simulink model "HFISaliencyTest"  (R2026b)
settings: Solver=ode4  StopTime=hfiTestCfg.Duration  FixedStep=hfiTestCfg.PlantStep
PostLoadFcn:
  | addpath(fullfile(fileparts(get_param(bdroot,'FileName')),'..','build_process'));initialize_hfi_probe_test(bdroot);
model workspace (MAT data in the model file):
  hfPlantCfg.Rs = 0.5
  hfPlantCfg.Ld = 0.001
  hfPlantCfg.Lq = 0.0015
  hfPlantCfg.Flux = 0.035
  hfPlantCfg.PolePairs = 4
  hfPlantCfg.J = 0.0005
  hfPlantCfg.B = 0.0001
  hfPlantCfg.Id0 = 0
  hfPlantCfg.Iq0 = 0
  hfPlantCfg.Speed0 = 0
  hfPlantCfg.Position0 = 0.175
  hfPlantCfg.SaturationDepth = 0
  hfPlantCfg.SaturationCurrent = 1
  hfPlantCfg.CrossInductance = 0
  hfPlantCfg.MechanicalEnabled = 1
  hfPlantCfg.Settings = [0.5; 0.001; 0.0015; 0.035; 4; 0.0005; 0.0001; 0; 1; 0; 1]
  hfPlantCfg.InitialState = [0; 0; 0; 0.175]
  hfiTestCfg.Duration = 0.05
  hfiTestCfg.Ts = 5e-05
  hfiTestCfg.PlantStep = 2.5e-06
  hfiTestCfg.InitialElectricalAngle = 0.7
  hfiTestCfg.InjectionScale = 1
  hfiTestCfg.Enable = 1
  hfiTestCfg.Reset = 0
  hfiTestCfg.LoadTorque = 0
  hfiTestCfg.MeasurementNoise = 0
  hfiTestCfg.NoiseSeed = 42
  hfiTestCfg.CurrentOffset = [0; 0; 0]
  hfiTestCfg.CurrentResolution = 0
  hfiTestCfg.CurrentRange = 8
  hfiTestCfg.CurrentDelay = 0
  hfiTestCfg.VoltageAlignmentDelay = 0
  hfiTestCfg.ExecutionDelay = 0
  hfiTestCfg.ActuationGain = 1
  hfiTestCfg.SaturationDepth = 0
  hfiTestCfg.CrossInductance = 0
  hfiTestCfg.MechanicalEnabled = 1
  probeCfg.Ts = 5e-05
  probeCfg.InjectionVoltage = 5
  probeCfg.WarmupSamples = 32
  probeCfg.CaptureSamples = 256
  probeCfg.MinSaliencyRatio = 0.08
  probeCfg.MaxSaliencyRatio = 0.8
  probeCfg.MinInverseInductance = 100
  probeCfg.MaxInverseInductance = 5000
  probeCfg.MaxFitResidual = 0.2
  probeCfg.MaxAsymmetry = 0.1
  probeCfg.MinVoltageRms = 1
  probeCfg.MaxCurrent = 2
  probeCfg.ProbeAxis = 0
  probeCfg.CrossPhase = 0
  probeCfg.Settings = [5e-05; 5; 32; 256; 0.08; 0.8; 100; 5000; 0.2; 0.1; 1; 2; 0; 0]
  probeCfg.InitialState = [0; 0; 0; 0; 0; 0; 0; 0; 0; 0; 0; 0; 0; 0; 0; 0; 0; 0; 0]
  testStim.time = [0 5e-05 0.0001 0.00015 0.0002 0.00025 0.0003 0.00035 0.0004 0.00045 0.0005 0.00055 ... (1001 elements, 1001x1)]
  testStim.signals.values = [0 0 0 0 0 0 0 0 0 0 0 0 ... (7007 elements, 1001x7)]
  testStim.signals.dimensions = 7
libraries: ClarkePark x2, PMSMHighFrequencyPlant x1, HighFrequencyObserver x1
settings Model: Creator=24322  LastModifiedBy=24322

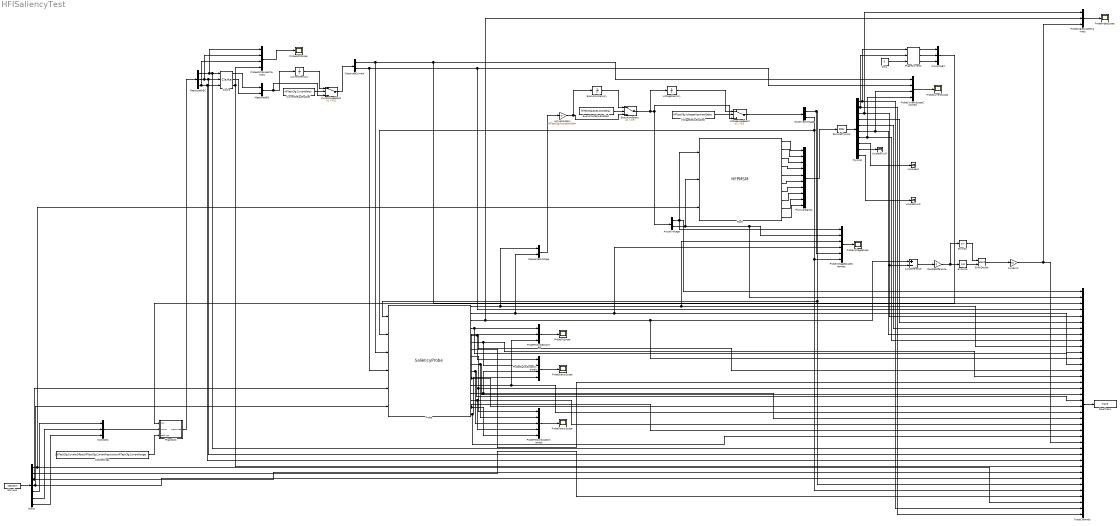
== system HFISaliencyTest ==
  ADCSettings : Constant  Value=[hfiTestCfg.CurrentOffset;hfiTestCfg.CurrentResolution;hfiTestCfg.CurrentRange]
  ActualVoltage : Demux  Outputs=2
  ActuationGain : Gain  Gain=hfiTestCfg.ActuationGain
  AxisDifference : Sum  Inputs=+-
  AxisError : Gain  Gain=0.5
  Clarke : ClarkePark/Clarke  SystemSampleTime=-1  VariantActivationTime=update diagram  EmptyChoice=off  PassThrough=off  PassThroughVariantControl=(default)  EmptyChoiceVariantControl=(default)  AllowFlexibleInterface=on  Latency=0  AutoFrameSizeCalculation=off
  CurrentABC : Mux  Inputs=3
  CurrentAgeSelect : Switch  Criteria=u2 > Threshold  Threshold=0.5  SaturateOnIntegerOverflow=off  InputSameDT=off
  CurrentDelayEnabled : Constant  Value=hfiTestCfg.CurrentDelay
  CurrentMemory : UnitDelay  InitialCondition=zeros(2,1)  SampleTime=probeCfg.Ts
  DoubleDifference : Gain  Gain=2
  ErrorCos : Trigonometry  Operator=cos
  ErrorDouble : Trigonometry  Operator=atan2
  ErrorSin : Trigonometry
  ExecutionDelayEnabled : Constant  Value=hfiTestCfg.ExecutionDelay
  ExecutionMemory : UnitDelay  InitialCondition=zeros(2,1)  SampleTime=probeCfg.Ts
  ExecutionSelect : Switch  Criteria=u2 > Threshold  Threshold=0.5  SaturateOnIntegerOverflow=off  InputSameDT=off
  Inputs : Demux  Outputs=7
  MeasuredAB : Mux  Inputs=2
  MeasuredABC : Demux  Outputs=3
  NoiseABC : Mux  Inputs=3
  ObservedCurrent : Demux  Outputs=2
  ObservedVoltage : Demux  Outputs=2
  PhaseADC : MATLAB Function  TreatAsAtomicUnit=on
  PhaseCurrents : ClarkePark/InverseClarke  SystemSampleTime=-1  VariantActivationTime=update diagram  EmptyChoice=off  PassThrough=off  PassThroughVariantControl=(default)  EmptyChoiceVariantControl=(default)  AllowFlexibleInterface=on  Latency=0  AutoFrameSizeCalculation=off
  Physical : Demux  Outputs=10
  PhysicalSignals : Mux  Inputs=10
  Plant : PMSMHighFrequencyPlant/HFPMSM  cfg=hfPlantCfg
  Probe : HighFrequencyObserver/SaliencyProbe  cfg=probeCfg
  ProbeADCScope : Scope
  ProbeADCScopeChannels : Mux
  ProbeAngleScope : Scope
  ProbeAngleScopeChannels : Mux  Inputs=3
  ProbeCurrentScope : Scope
  ProbeCurrentScopeChannels : Mux
  ProbeFitScope : Scope
  ProbeFitScopeChannels : Mux  Inputs=3
  ProbeStatusScope : Scope
  ProbeStatusScopeChannels : Mux
  ProbeTensorScope : Scope
  ProbeTensorScopeChannels : Mux  Inputs=5
  ProbeVoltageScope : Scope
  ProbeVoltageScopeChannels : Mux  Inputs=6
  RequestedVoltage : Mux  Inputs=2
  SamplePhysical : ZeroOrderHold  SampleTime=probeCfg.Ts
  SaveTrace : ToWorkspace  VariableName=trace  SaveFormat=Structure With Time  SampleTime=-1
  Stimulus : FromWorkspace  VariableName=testStim  SampleTime=probeCfg.Ts  Interpolate=off  OutputAfterFinalValue=Holding final value
  TraceChannels : Mux  Inputs=38
  UnusedFluxD : Terminator
  UnusedFluxQ : Terminator
  UnusedLd : Terminator
  VoltageAgeSelect : Switch  Criteria=u2 > Threshold  Threshold=0.5  SaturateOnIntegerOverflow=off  InputSameDT=off
  VoltageDelayEnabled : Constant  Value=hfiTestCfg.VoltageAlignmentDelay
  VoltageMemory : UnitDelay  InitialCondition=zeros(2,1)  SampleTime=probeCfg.Ts
  Zero : Constant  Value=0
  wires:
  Stimulus/1 -> Inputs/1
  RequestedVoltage/1 -> ActuationGain/1
  ActuationGain/1 -> ExecutionMemory/1, ExecutionSelect/3
  ExecutionMemory/1 -> ExecutionSelect/1
  ExecutionDelayEnabled/1 -> ExecutionSelect/2
  ExecutionSelect/1 -> ActualVoltage/1, VoltageAgeSelect/3, VoltageMemory/1
  VoltageMemory/1 -> VoltageAgeSelect/1
  VoltageDelayEnabled/1 -> VoltageAgeSelect/2
  VoltageAgeSelect/1 -> ObservedVoltage/1
  PhysicalSignals/1 -> SamplePhysical/1
  SamplePhysical/1 -> Physical/1
  CurrentABC/1 -> PhaseADC/1(raw)
  NoiseABC/1 -> PhaseADC/2(noise)
  ADCSettings/1 -> PhaseADC/3(settings)
  PhaseADC/1(measured) -> MeasuredABC/1
  MeasuredAB/1 -> CurrentAgeSelect/3, CurrentMemory/1
  CurrentMemory/1 -> CurrentAgeSelect/1
  CurrentDelayEnabled/1 -> CurrentAgeSelect/2
  CurrentAgeSelect/1 -> ObservedCurrent/1
  Zero/1 -> PhaseCurrents/3
  AxisDifference/1 -> DoubleDifference/1
  DoubleDifference/1 -> ErrorSin/1, ErrorCos/1
  ErrorSin/1 -> ErrorDouble/1
  ErrorCos/1 -> ErrorDouble/2
  ErrorDouble/1 -> AxisError/1
  TraceChannels/1 -> SaveTrace/1
  Inputs/1 -> TraceChannels/36, Plant/3
  Inputs/3 -> TraceChannels/31, Probe/5
  Inputs/4 -> TraceChannels/32, Probe/6
  Physical/1 -> PhaseCurrents/1, TraceChannels/37
  Physical/2 -> PhaseCurrents/2, TraceChannels/38
  Probe/3 -> TraceChannels/12, AxisDifference/1, ProbeAngleScopeChannels/2
  Physical/3 -> AxisDifference/2, TraceChannels/5, ProbeAngleScopeChannels/1
  Physical/8 -> UnusedLd/1
  Physical/9 -> UnusedFluxD/1
  Physical/10 -> UnusedFluxQ/1
  Probe/1 -> ProbeVoltageScopeChannels/3, TraceChannels/10, RequestedVoltage/1
  ActualVoltage/1 -> TraceChannels/1, ProbeVoltageScopeChannels/1, Plant/1
  ObservedVoltage/1 -> TraceChannels/33, Probe/1, ProbeVoltageScopeChannels/5
  ObservedCurrent/1 -> TraceChannels/3, ProbeCurrentScopeChannels/1, Probe/3
  Clarke/1 -> MeasuredAB/1
  Probe/2 -> ProbeVoltageScopeChannels/4, TraceChannels/11, RequestedVoltage/2
  ActualVoltage/2 -> ProbeVoltageScopeChannels/2, TraceChannels/2, Plant/2
  ObservedVoltage/2 -> TraceChannels/34, ProbeVoltageScopeChannels/6, Probe/2
  ObservedCurrent/2 -> TraceChannels/4, ProbeCurrentScopeChannels/2, Probe/4
  Clarke/2 -> MeasuredAB/2
  PhaseCurrents/1 -> CurrentABC/1
  MeasuredABC/1 -> TraceChannels/27, Clarke/1, ProbeADCScopeChannels/1
  Inputs/5 -> NoiseABC/1
  PhaseCurrents/2 -> CurrentABC/2
  MeasuredABC/2 -> TraceChannels/28, Clarke/2, ProbeADCScopeChannels/2
  Inputs/6 -> NoiseABC/2
  PhaseCurrents/3 -> CurrentABC/3
  MeasuredABC/3 -> TraceChannels/29, Clarke/3, ProbeADCScopeChannels/3
  Inputs/7 -> NoiseABC/3
  Plant/1 -> PhysicalSignals/1
  Plant/2 -> PhysicalSignals/2
  Plant/3 -> PhysicalSignals/3
  Plant/4 -> PhysicalSignals/4
  Plant/5 -> PhysicalSignals/5
  Plant/6 -> PhysicalSignals/6
  Plant/7 -> PhysicalSignals/7
  Plant/8 -> PhysicalSignals/8
  Plant/9 -> PhysicalSignals/9
  Plant/10 -> PhysicalSignals/10
  Physical/4 -> TraceChannels/6
  Physical/5 -> TraceChannels/7
  Physical/6 -> TraceChannels/8, ProbeCurrentScopeChannels/3
  Physical/7 -> TraceChannels/9, ProbeCurrentScopeChannels/4
  Probe/4 -> TraceChannels/13, ProbeFitScopeChannels/1
  Probe/5 -> TraceChannels/14, ProbeStatusScopeChannels/1
  Probe/6 -> TraceChannels/15, ProbeStatusScopeChannels/2
  Probe/7 -> TraceChannels/16
  Probe/8 -> TraceChannels/17, ProbeTensorScopeChannels/1
  Probe/9 -> ProbeTensorScopeChannels/2, TraceChannels/18
  Probe/10 -> ProbeTensorScopeChannels/3, TraceChannels/19
  Probe/11 -> TraceChannels/20, ProbeFitScopeChannels/2
  Probe/12 -> TraceChannels/21, ProbeFitScopeChannels/3
  Probe/13 -> TraceChannels/22, ProbeStatusScopeChannels/3
  Probe/14 -> ProbeTensorScopeChannels/4, TraceChannels/23
  Probe/15 -> ProbeTensorScopeChannels/5, TraceChannels/24
  Probe/16 -> TraceChannels/25, ProbeStatusScopeChannels/4
  AxisError/1 -> ProbeAngleScopeChannels/3, TraceChannels/26
  Clarke/3 -> TraceChannels/30, ProbeADCScopeChannels/4
  Inputs/2 -> TraceChannels/35
  ProbeAngleScopeChannels/1 -> ProbeAngleScope/1
  ProbeTensorScopeChannels/1 -> ProbeTensorScope/1
  ProbeStatusScopeChannels/1 -> ProbeStatusScope/1
  ProbeFitScopeChannels/1 -> ProbeFitScope/1
  ProbeVoltageScopeChannels/1 -> ProbeVoltageScope/1
  ProbeCurrentScopeChannels/1 -> ProbeCurrentScope/1
  ProbeADCScopeChannels/1 -> ProbeADCScope/1

== matlab function HFISaliencyTest/PhaseADC ==
  data: raw input; measured output; noise input; settings input
function measured=hfi_measure_current(raw,noise,settings)
%HFI_MEASURE_CURRENT Three phase ADC fixture: offset, noise, clipping, rounding.
% settings=[offset_a;offset_b;offset_c;resolution_A;range_A].
%#codegen
measured=min(max(raw+noise+settings(1:3),-settings(5)),settings(5));
if settings(4)>0
    measured=round(measured/settings(4))*settings(4);
end
end
